simulink library "Lib_Piccolo"  (R2018b)
settings: Solver=VariableStepAuto  StartTime=0.0  StopTime=10.0  RelTol=1e-3
values from neighbouring files (symbols this model uses):
  AccelErrInt2Brakes = 0.15    [SimulationControlConfig16P.m]    (also in SimulationControlConfig16P_LEGACY.m; SimulationControlConfigTAILLESS.m = 0.2; SimulationControlConfigUTAIL.m = 0.2)
  AileronMax = 25    [SimulationControlConfig16P.m]    (also in SimulationControlConfig16P_LEGACY.m; SimulationControlConfigTAILLESS.m; SimulationControlConfigUTAIL.m)
  AileronPower = 0.00268    [SimulationControlConfig16P.m]    (also in SimulationControlConfig16P_LEGACY.m; SimulationControlConfigTAILLESS.m; SimulationControlConfigUTAIL.m)
  AileronSurfaceMax = 45    [SimulationControlConfig16P.m]    (also in SimulationControlConfig16P_LEGACY.m)
  AileronTrim = 0    [SimulationControlConfig16P.m]    (also in SimulationControlConfig16P_LEGACY.m; SimulationControlConfigTAILLESS.m; SimulationControlConfigUTAIL.m)
  Alt = 1000 + TerrainHeight    [SimulationStateConfig.m]
  AltCruise_m = testPlans(testIndx).terrainElevation * 0.3048 + 200    [SimulationControlConfig16P.m]    (also in SimulationControlConfigTAILLESS.m = 1083; SimulationControlConfigUTAIL.m = testPlans(testIndx).terrainElevation * 0.3048 + 152)
  AltitudeRate2PitchCmdIntegratorInit = 0.1    [SimulationControlPre.m]
  AltMax = 10000    [SimulationControlConfig16P.m]    (also in SimulationControlConfig16P_LEGACY.m; SimulationControlConfigTAILLESS.m; SimulationControlConfigUTAIL.m)
  AltMaxAccel = 1.25    [SimulationControlConfig16P.m]    (also in SimulationControlConfig16P_LEGACY.m = 0.9; SimulationControlConfigTAILLESS.m = 1.7; SimulationControlConfigUTAIL.m = 2)
  AltMin = 0    [SimulationControlConfig16P.m]    (also in SimulationControlConfig16P_LEGACY.m; SimulationControlConfigTAILLESS.m; SimulationControlConfigUTAIL.m)
  AltRateCmd2Pitch = 0.50    (= 0.5)    [SimulationControlConfig16P.m]    (also in SimulationControlConfig16P_LEGACY.m = 0.6; SimulationControlConfigTAILLESS.m = 0.2; SimulationControlConfigUTAIL.m = 0.3)
  AltRateError2Pitch = 0.40    (= 0.4)    [SimulationControlConfig16P.m]    (also in SimulationControlConfig16P_LEGACY.m; SimulationControlConfigTAILLESS.m = 0.55; SimulationControlConfigUTAIL.m = 0.55)
  AltRateErrorInt2Pitch = 0.50    (= 0.5)    [SimulationControlConfig16P.m]    (also in SimulationControlConfig16P_LEGACY.m = 0.45; SimulationControlConfigTAILLESS.m; SimulationControlConfigUTAIL.m = 0.75)
  AltRateLpfCutOff = 3    [SimulationControlConfig16P.m]    (also in SimulationControlConfig16P_LEGACY.m; SimulationControlConfigTAILLESS.m = 2; SimulationControlConfigUTAIL.m = 2)
  AutoNosegear2Rudder = 26    [SimulationControlConfig16P.m]    (also in SimulationControlConfig16P_LEGACY.m; SimulationControlConfigTAILLESS.m = 25.2; SimulationControlConfigUTAIL.m = 14)
  b = 5.54    [SimulationControlConfig16P.m]    (also in SimulationControlConfig16P_LEGACY.m; SimulationControlConfigTAILLESS.m = 2.37; SimulationControlConfigUTAIL.m = 2.37)
  Bank2AileronIntegratorInit = 0    [SimulationControlPre.m]
  BankMax_User = BankMax_User/180*pi    (= 0.523598775598)    [SimulationControlConfig16P.m]    (also in SimulationControlConfig16P_LEGACY.m; SimulationControlConfigTAILLESS.m = 0.610865238198; SimulationControlConfigUTAIL.m = 0.628318530718)
  baseLegFlaps = 20    [SimulationControlConfig16P.m]    (also in SimulationControlConfig16P_LEGACY.m = 0; SimulationControlConfigTAILLESS.m = 15; SimulationControlConfigUTAIL.m = 10)
  C = GeneticOpt.C    [SimulationCostFunction.m]
  c = Sw/b    (= 0.841696750903)    [SimulationControlConfig16P.m]    (also in SimulationControlConfig16P_LEGACY.m; SimulationControlConfigTAILLESS.m = 0.354008438819; SimulationControlConfigUTAIL.m = 0.354008438819)
  cell2WheelFactorMG = 5.98    [SimulationSensorConfig16P_LEGACY.m]
  cell2WheelFactorNG = 1    [SimulationSensorConfig16P_LEGACY.m]
  cellSatMaxMG = 15000    [SimulationSensorConfig16P.m]    (also in SimulationSensorConfig16P_LEGACY.m; SimulationSensorConfigTAILLESS7P.m; SimulationSensorConfigUTAIL7P.m)
  cellSatMaxNG = 1000    [SimulationSensorConfig16P.m]    (also in SimulationSensorConfig16P_LEGACY.m; SimulationSensorConfigTAILLESS7P.m; SimulationSensorConfigUTAIL7P.m)
  cellSatMinMG = -15000    [SimulationSensorConfig16P.m]    (also in SimulationSensorConfig16P_LEGACY.m; SimulationSensorConfigTAILLESS7P.m; SimulationSensorConfigUTAIL7P.m)
  cellSatMinNG = -1000    [SimulationSensorConfig16P.m]    (also in SimulationSensorConfig16P_LEGACY.m; SimulationSensorConfigTAILLESS7P.m; SimulationSensorConfigUTAIL7P.m)
  CL_Limit = CL_Max    (= 0.54)    [SimulationControlConfig16P.m]    (also in SimulationControlConfig16P_LEGACY.m; SimulationControlConfigTAILLESS.m; SimulationControlConfigUTAIL.m = 0.53)
  CL_Max = 0.54    [SimulationControlConfig16P.m]    (also in SimulationControlConfig16P_LEGACY.m; SimulationControlConfigTAILLESS.m; SimulationControlConfigUTAIL.m = 0.53)
  CL_Max_Nom = 0.465    [SimulationControlConfig16P.m]    (also in SimulationControlConfig16P_LEGACY.m; SimulationControlConfigTAILLESS.m = 0.39; SimulationControlConfigUTAIL.m)
  CL_Min = 0    [SimulationControlConfig16P.m]    (also in SimulationControlConfig16P_LEGACY.m; SimulationControlConfigTAILLESS.m; SimulationControlConfigUTAIL.m)
  ClimbMaxFraction = 0.35    [SimulationControlConfig16P.m]    (also in SimulationControlConfig16P_LEGACY.m = 0.24; SimulationControlConfigTAILLESS.m = 0.19; SimulationControlConfigUTAIL.m = 0.21)
  ClimboutMaxBank = 7.0    (= 7)    [SimulationControlConfig16P.m]    (also in SimulationControlConfig16P_LEGACY.m; SimulationControlConfigTAILLESS.m = 5; SimulationControlConfigUTAIL.m)
  ClimboutTimer = 7.0    (= 7)    [SimulationControlConfig16P.m]    (also in SimulationControlConfig16P_LEGACY.m; SimulationControlConfigTAILLESS.m; SimulationControlConfigUTAIL.m)
  dCl_per_dFlap = 0.005581818    [SimulationControlConfig16P.m]    (also in SimulationControlConfig16P_LEGACY.m = 0; SimulationControlConfigTAILLESS.m = 0; SimulationControlConfigUTAIL.m = 0)
  DecelerationCmd = 3.1    [SimulationControlConfig16P.m]    (also in SimulationControlConfig16P_LEGACY.m; SimulationControlConfigTAILLESS.m = 0.1; SimulationControlConfigUTAIL.m = 0.1)
  DeRotateLogicEndTimer = abs((NoseDownLimit_Deg-1)/DeRotateRamp_Dps)    [SimulationControlConfig16P.m]    (also in SimulationControlConfig16P_LEGACY.m; SimulationControlConfigTAILLESS.m; SimulationControlConfigUTAIL.m)
  DeRotateLogicHoldNoseUpTimer = 0.1    [SimulationControlConfig16P.m]    (also in SimulationControlConfig16P_LEGACY.m; SimulationControlConfigTAILLESS.m; SimulationControlConfigUTAIL.m)
  DeRotateLogicTimerTimeout = 2    [SimulationControlConfig16P.m]    (also in SimulationControlConfig16P_LEGACY.m; SimulationControlConfigTAILLESS.m; SimulationControlConfigUTAIL.m)
  DeRotateLowerCmdSaturation = 0    [SimulationControlConfig16P.m]    (also in SimulationControlConfig16P_LEGACY.m; SimulationControlConfigTAILLESS.m; SimulationControlConfigUTAIL.m)
  DeRotateRamp_Dps = 3    [SimulationControlConfig16P.m]    (also in SimulationControlConfig16P_LEGACY.m; SimulationControlConfigTAILLESS.m = 8; SimulationControlConfigUTAIL.m = 8)
  DeRotateUpperCmdSaturation = 7    [SimulationControlConfig16P.m]    (also in SimulationControlConfig16P_LEGACY.m; SimulationControlConfigTAILLESS.m; SimulationControlConfigUTAIL.m)
  DescentMaxFraction = 0.22    [SimulationControlConfig16P.m]    (also in SimulationControlConfig16P_LEGACY.m = 0.2; SimulationControlConfigTAILLESS.m = 0.17; SimulationControlConfigUTAIL.m = 0.17)
  DesktopSimTerrainOffset_m = 0.406    [SimulationAircraftConfig.m]
  downwindFlaps = 0    [SimulationControlConfig16P.m]    (also in SimulationControlConfig16P_LEGACY.m; SimulationControlConfigTAILLESS.m; SimulationControlConfigUTAIL.m)
  DP_init = 0.5*1.225*V_init^2    [SimulationControlConfig16P.m]    (also in SimulationControlConfig16P_LEGACY.m; SimulationControlConfigTAILLESS.m; SimulationControlConfigUTAIL.m)
  dscNoiseMG = 1    [SimulationSensorConfig16P_LEGACY.m]
  dscNoiseNG = 0.25    [SimulationSensorConfig16P_LEGACY.m]
  DSCnumBits = 24    [SimulationSensorConfig16P.m]    (also in SimulationSensorConfig16P_LEGACY.m; SimulationSensorConfigTAILLESS7P.m; SimulationSensorConfigUTAIL7P.m)
  DSCRangeMaxMG = 15000    [SimulationSensorConfig16P.m]    (also in SimulationSensorConfig16P_LEGACY.m; SimulationSensorConfigTAILLESS7P.m; SimulationSensorConfigUTAIL7P.m)
  DSCRangeMaxNG = 1000    [SimulationSensorConfig16P.m]    (also in SimulationSensorConfig16P_LEGACY.m; SimulationSensorConfigTAILLESS7P.m; SimulationSensorConfigUTAIL7P.m)
  DSCRangeMinMG = -15000    [SimulationSensorConfig16P.m]    (also in SimulationSensorConfig16P_LEGACY.m; SimulationSensorConfigTAILLESS7P.m; SimulationSensorConfigUTAIL7P.m)
  DSCRangeMinNG = -1000    [SimulationSensorConfig16P.m]    (also in SimulationSensorConfig16P_LEGACY.m; SimulationSensorConfigTAILLESS7P.m; SimulationSensorConfigUTAIL7P.m)
  dt = DLLSim.dt    [SimulationTimeStep.m]    (also in SimulationTrim.m = 0.02)
  EarlyTouchdownThreshold = 3.0    (= 3)    [SimulationControlConfig16P.m]    (also in SimulationControlConfig16P_LEGACY.m; SimulationControlConfigTAILLESS.m = 2.2; SimulationControlConfigUTAIL.m = 2.5)
  ElevatorDeflectionRate = 15    [SimulationControlConfig16P.m]    (also in SimulationControlConfig16P_LEGACY.m = 12; SimulationControlConfigTAILLESS.m = 10; SimulationControlConfigUTAIL.m = 12)
  ElevatorMax = 25    [SimulationControlConfig16P.m]    (also in SimulationControlConfig16P_LEGACY.m; SimulationControlConfigTAILLESS.m; SimulationControlConfigUTAIL.m)
  ElevatorPower = -0.002209    [SimulationControlConfig16P.m]    (also in SimulationControlConfig16P_LEGACY.m; SimulationControlConfigTAILLESS.m = -0.002956; SimulationControlConfigUTAIL.m = -0.00205983)
  ElevatorTrim = -3.5    [SimulationControlConfig16P.m]    (also in SimulationControlConfig16P_LEGACY.m; SimulationControlConfigTAILLESS.m = -6; SimulationControlConfigUTAIL.m = -8)
  elevonBias = 0    [SimulationControlConfig16P.m]    (also in SimulationControlConfig16P_LEGACY.m; SimulationControlConfigTAILLESS.m; SimulationControlConfigUTAIL.m)
  Enable_TAS_Protection = 0    [SimulationControlConfig16P.m]    (also in SimulationControlConfig16P_LEGACY.m; SimulationControlConfigTAILLESS.m; SimulationControlConfigUTAIL.m)
  EnableCrossTrackAbort = 1    [SimulationControlConfig16P.m]    (also in SimulationControlConfigTAILLESS.m; SimulationControlConfigUTAIL.m)
  EnergyBandwidth = 0.02    [SimulationControlConfig16P.m]    (also in SimulationControlConfig16P_LEGACY.m; SimulationControlConfigTAILLESS.m = 0.06; SimulationControlConfigUTAIL.m = 0.06)
  EngineLhFuelCut = 0    [SimulationAircraftConfig.m]
  EngineRhFuelCut = 0    [SimulationAircraftConfig.m]
  FastThrottleRate = 0.075    [SimulationControlConfig16P.m]    (also in SimulationControlConfig16P_LEGACY.m = 0.05; SimulationControlConfigTAILLESS.m = 0.1; SimulationControlConfigUTAIL.m = 0.1)
  FilterWarmUpTime = 2    [SimulationSensorConfig16P.m]    (also in SimulationSensorConfig16P_LEGACY.m; SimulationSensorConfigTAILLESS7P.m; SimulationSensorConfigUTAIL7P.m)
  finalApproachFlaps = 20    [SimulationControlConfig16P.m]    (also in SimulationControlConfig16P_LEGACY.m = 0; SimulationControlConfigTAILLESS.m = 22; SimulationControlConfigUTAIL.m = 10)
  FinalDescentSlope_Deg = testPlans(testIndx).descentSlope    [SimulationControlConfig16P.m]    (also in SimulationControlConfig16P_LEGACY.m; SimulationControlConfigTAILLESS.m; SimulationControlConfigUTAIL.m)
  flapMax = 0    [SimulationControlConfig16P.m]    (also in SimulationControlConfig16P_LEGACY.m; SimulationControlConfigTAILLESS.m; SimulationControlConfigUTAIL.m)
  flapRate = 7.5    [SimulationControlConfig16P.m]    (also in SimulationControlConfig16P_LEGACY.m; SimulationControlConfigTAILLESS.m = 6.6; SimulationControlConfigUTAIL.m)
  FlareHeight = 5    [SimulationControlConfig16P.m]    (also in SimulationControlConfig16P_LEGACY.m = 4.8; SimulationControlConfigTAILLESS.m = 2.5; SimulationControlConfigUTAIL.m = 2)
  FlareVerticalRate_mps = -0.4    [SimulationControlConfig16P.m]    (also in SimulationControlConfig16P_LEGACY.m = -0.5; SimulationControlConfigTAILLESS.m = -0.15; SimulationControlConfigUTAIL.m = -0.15)
  Fp_Aileron = 0.55*2*pi*RollRateLpfCutoff*dt    [SimulationControlConfig16P.m]    (also in SimulationControlConfig16P_LEGACY.m; SimulationControlConfigTAILLESS.m; SimulationControlConfigUTAIL.m)
  Fp_Alt = 0.55*AltBandwidth    (= 0.099)    [SimulationControlConfig16P.m]    (also in SimulationControlConfig16P_LEGACY.m; SimulationControlConfigTAILLESS.m = 0.587477826221; SimulationControlConfigUTAIL.m = 0.69115038379)
  Fp_AltRate = 0.55*2*pi*AltRateLpfCutOff*dt    [SimulationControlConfig16P.m]    (also in SimulationControlConfig16P_LEGACY.m; SimulationControlConfigTAILLESS.m; SimulationControlConfigUTAIL.m)
  Fp_Elevator = 0.55*2*pi*PitchRateLpfCutoff*dt    [SimulationControlConfig16P.m]    (also in SimulationControlConfig16P_LEGACY.m; SimulationControlConfigTAILLESS.m; SimulationControlConfigUTAIL.m)
  Fp_Energy = 0.55*2*pi*EnergyBandwidth    (= 0.069115038379)    [SimulationControlConfig16P.m]    (also in SimulationControlConfig16P_LEGACY.m; SimulationControlConfigTAILLESS.m = 0.207345115137; SimulationControlConfigUTAIL.m = 0.207345115137)
  Fp_Energy2 = 0.55*2*pi*EnergyBandwidth*dt    [SimulationControlConfig16P.m]    (also in SimulationControlConfig16P_LEGACY.m; SimulationControlConfigTAILLESS.m; SimulationControlConfigUTAIL.m)
  Fp_Pitch = 0.55*2*pi*PitchBandwidth    (= 2.76460153516)    [SimulationControlConfig16P.m]    (also in SimulationControlConfig16P_LEGACY.m = 3.11017672705; SimulationControlConfigTAILLESS.m = 3.80132711084; SimulationControlConfigUTAIL.m = 2.41902634326)
  Fp_Pitch_2 = 0.55*2*pi*PitchBandwidth*dt    [SimulationControlConfig16P.m]    (also in SimulationControlConfig16P_LEGACY.m; SimulationControlConfigTAILLESS.m; SimulationControlConfigUTAIL.m)
  Fp_Roll = RollBandwidth^2    (= 1)    [SimulationControlConfig16P.m]    (also in SimulationControlConfig16P_LEGACY.m = 1.44; SimulationControlConfigTAILLESS.m; SimulationControlConfigUTAIL.m)
  Fp_Rudder = 0.55*2*pi*YawRateLpfCutoff*dt    [SimulationControlConfig16P.m]    (also in SimulationControlConfig16P_LEGACY.m; SimulationControlConfigTAILLESS.m; SimulationControlConfigUTAIL.m)
  Fp_TAS = 0.55*2*pi*TASBandwidth    (= 0.103672557568)    [SimulationControlConfig16P.m]    (also in SimulationControlConfig16P_LEGACY.m; SimulationControlConfigTAILLESS.m = 0.172787595947; SimulationControlConfigUTAIL.m = 0.172787595947)
  Fp_TAS_Filter = 2*pi*TasLpfCutoff*dt    [SimulationControlConfig16P.m]    (also in SimulationControlConfig16P_LEGACY.m; SimulationControlConfigTAILLESS.m; SimulationControlConfigUTAIL.m)
  Fp_Turn = 0.55*2*pi*TurnErrLPFcutoff    (= 0.0345575191895)    [SimulationControlConfig16P.m]    (also in SimulationControlConfig16P_LEGACY.m; SimulationControlConfigTAILLESS.m = 0.172787595947; SimulationControlConfigUTAIL.m = 0.172787595947)
  Fp_TurnDerr = 0.55*2*pi*TurnDerivativeLPFcutoff    (= 0.0345575191895)    [SimulationControlConfig16P.m]    (also in SimulationControlConfig16P_LEGACY.m; SimulationControlConfigTAILLESS.m = 0.172787595947; SimulationControlConfigUTAIL.m = 0.172787595947)
  FTV = 3    [SimulationAircraftConfig.m]
  ftvStaticPositionError = 1/1.18    (= 0.847457627119)    [SimulationSensorConfig16P.m]    (also in SimulationSensorConfig16P_LEGACY.m; SimulationSensorConfigTAILLESS7P.m = 1; SimulationSensorConfigUTAIL7P.m = 1)
  g = 9.81    [SimulationStateConfig.m]
  GustSpd_Kts = testPlans(testIndx).gustSpd    [SimulationStateConfig.m]
  GustTriggerVal = testPlans(testIndx).gustTriggerVal    [SimulationStateConfig.m]
  HeadingErr2TurnRate = 0.5    [SimulationControlConfig16P.m]    (also in SimulationControlConfig16P_LEGACY.m; SimulationControlConfigTAILLESS.m; SimulationControlConfigUTAIL.m)
  HeadingErrDer2TurnRate = 0.3    [SimulationControlConfig16P.m]    (also in SimulationControlConfig16P_LEGACY.m; SimulationControlConfigTAILLESS.m; SimulationControlConfigUTAIL.m)
  IASbounce = IASstall*0.8    [SimulationControlPre.m]
  IAScruiseCMD = sqrt(2*m*9.81/(1.225*Sw*CL_cruise))    [SimulationControlConfig16P.m]    (also in SimulationControlConfig16P_LEGACY.m; SimulationControlConfigTAILLESS.m; SimulationControlConfigUTAIL.m)
  IASfinalCMD = 1.12 * IASmin    [SimulationControlConfig16P.m]    (also in SimulationControlConfig16P_LEGACY.m = 1.10 * IASmin; SimulationControlConfigTAILLESS.m = 1.10 * IASmin; SimulationControlConfigUTAIL.m = 1.15 * IASmin)
  IASflareCMD = IASstall    [SimulationControlConfig16P.m]    (also in SimulationControlConfig16P_LEGACY.m; SimulationControlConfigTAILLESS.m; SimulationControlConfigUTAIL.m)
  IASmax = 64    [SimulationControlConfig16P.m]    (also in SimulationControlConfig16P_LEGACY.m = 46; SimulationControlConfigTAILLESS.m = 38.58; SimulationControlConfigUTAIL.m = 35)
  IASmin = sqrt(2*m*9.81/(1.225*Sw*0.9*CL_Max_Nom))    [SimulationControlConfig16P.m]    (also in SimulationControlConfig16P_LEGACY.m; SimulationControlConfigTAILLESS.m; SimulationControlConfigUTAIL.m)
  IASshortCMD = IASstall    [SimulationControlConfig16P.m]    (also in SimulationControlConfig16P_LEGACY.m; SimulationControlConfigTAILLESS.m; SimulationControlConfigUTAIL.m)
  IASstall = sqrt(2*m*9.81/(1.225*Sw*CL_Max))    [SimulationControlConfig16P.m]    (also in SimulationControlConfig16P_LEGACY.m; SimulationControlConfigTAILLESS.m; SimulationControlConfigUTAIL.m)
  inFlight = 1    [SimulationControlConfig16P.m]    (also in SimulationControlConfigTAILLESS.m; SimulationControlConfigUTAIL.m)
  JetCatOffset = 5    [SimulationControlConfig16P.m]    (also in SimulationControlConfig16P_LEGACY.m)
  LaunchRollingElevator = -1.5    [SimulationControlConfig16P.m]    (also in SimulationControlConfig16P_LEGACY.m; SimulationControlConfigTAILLESS.m = 1; SimulationControlConfigUTAIL.m = 1)
  ldg_NosegearMax = 10    [SimulationControlConfig16P.m]    (also in SimulationControlConfig16P_LEGACY.m; SimulationControlConfigTAILLESS.m; SimulationControlConfigUTAIL.m)
  ldg_TrackVyErrInt2Nosegear = 0.1250    (= 0.125)    [SimulationControlConfig16P.m]    (also in SimulationControlConfig16P_LEGACY.m; SimulationControlConfigTAILLESS.m = 0.00714285714286; SimulationControlConfigUTAIL.m = 0.00714285714286)
  ldg_TrackVyErrPro2Nosegear = 0.35    [SimulationControlConfig16P.m]    (also in SimulationControlConfig16P_LEGACY.m; SimulationControlConfigTAILLESS.m = 0.0546666666667; SimulationControlConfigUTAIL.m = 0.0546666666667)
  ldg_TrackY2Vy = 0.07    [SimulationControlConfig16P.m]    (also in SimulationControlConfig16P_LEGACY.m; SimulationControlConfigTAILLESS.m = 0.17; SimulationControlConfigUTAIL.m = 0.17)
  ldg_Vy2NosegearScalingPower = 1.075    [SimulationControlConfig16P.m]    (also in SimulationControlConfig16P_LEGACY.m; SimulationControlConfigTAILLESS.m = 0.6; SimulationControlConfigUTAIL.m = 0.5)
  ldg_Y2VyScalingPower = 0.175    [SimulationControlConfig16P.m]    (also in SimulationControlConfig16P_LEGACY.m; SimulationControlConfigTAILLESS.m = 0; SimulationControlConfigUTAIL.m = 0)
  ldg_YawRate2Nosegear = 0.175    [SimulationControlConfig16P.m]    (also in SimulationControlConfig16P_LEGACY.m; SimulationControlConfigTAILLESS.m = 0.065; SimulationControlConfigUTAIL.m = 0.065)
  LiftSlope = 0.064285    [SimulationControlConfig16P.m]    (also in SimulationControlConfig16P_LEGACY.m; SimulationControlConfigTAILLESS.m = 0.058631; SimulationControlConfigUTAIL.m)
  LPFaileronInit = 0    [SimulationControlPre.m]
  LPFclestInit = 0    [SimulationControlPre.m]
  LPFenergyFFInit = 0    [SimulationControlPre.m]
  LPFtasInit = V_init + 2    [SimulationControlPre.m]
  LPFthrottleInit = ThrottleTrim    [SimulationControlPre.m]
  LPFturnErrInit = 0    [SimulationControlPre.m]
  ... (+115 more)
undefined symbols (not defined in the file or in its folder): abortFlag, alphaHPF, apmDelay, BRWNOUT, CRAWOR, CRAWUR, DiscIntNeverNeededParam, DLLSim, DLLSimStep, ECOMOR, ECOMUR, Fp_Tas, GustTrigger_HeightAgl_m, IPSTAT, LCINTEG, Ldg_Persist_Time, LOWER_FLAGS, MSG_ENABLE, NoiseStd, OLDVAL, OVERRIDE_ENABLE, OVERRIDE_VALUE, REBOOT, reversionEnable, revIASMax, revIASMin, revPitchMax, revPitchMin, revPitchRateMax, revRollMax, revRollRateMax, SAMPLE, SCALON, SensorModel, sigbuilder_block, Sim_Vx, Sim_Vy, Sim_Vz, Sim_Xpos, Sim_Ypos, Sim_Zpos, SYSOR, SYSUR, TARE, TEMPOR, TEMPUR, testIndx, testPlan, testPlans, Trim_piccoloInCmd, Trim_REFSI_FD_IN_nmodeCgShifterCmd_Ft, Trim_REFSI_FD_IN_nmodeFlapLhIBCmd_Deg, Trim_REFSI_FD_IN_nmodeFlapLhOBCmd_Deg, Trim_REFSI_FD_IN_nmodeFlapRhIBCmd_Deg, Trim_REFSI_FD_IN_nmodeFlapRhOBCmd_Deg, Trim_REFSI_FD_IN_nmodeSlatLhCmd_Deg, Trim_REFSI_FD_IN_nmodeSlatRhCmd_Deg, Trim_REFSI_FD_IN_nmodeSplrLhInbdCmd_Deg, Trim_REFSI_FD_IN_nmodeSplrLhOutbdCmd_Deg ... (+5)
libraries: simulink x866, aerolibconvert2 x60, $bdroot x52, aerolibatmos2 x5, dspswit3 x5, simulink_extras x4, dsparch4 x2, Lib_Piccolo_Alt x2, eeGeneralControl x1, dspindex x1
(part 34 of 44)

== system Lib_Piccolo/Ground Detection Systems/WoW Wrapper/Variant Subsystem/Load Cell WoW Model 1 7P AsFlown/LPF N ==
  Input : Inport
  Reset : Inport  Port=2
  Add1 : Sum  Inputs=++|
  Compare To Constant2 : simulink/Logic and Bit Operations/Compare To Constant  relop=>  const=0  OutDataTypeStr=uint8
  Constant11 : Constant  Value=2
  Switch1 : Switch  Criteria=u2 > Threshold
  Unit Delay1 : UnitDelay  InitialCondition=Init  SampleTime=-1
  a1 : Gain  Gain=1-0.221168
  b0 : Gain  Gain=0.221168
  Output : Outport
  wires:
  Constant11/1 -> Compare To Constant2/1
  Compare To Constant2/1 -> Switch1/2
  Switch1/1 -> Output/1
  Input/1 -> b0/1, Switch1/3
  a1/1 -> Add1/1
  Add1/1 -> Switch1/1, Unit Delay1/1
  b0/1 -> Add1/2
  Unit Delay1/1 -> a1/1

== system Lib_Piccolo/Ground Detection Systems/WoW Wrapper/Variant Subsystem/Load Cell WoW Model 1 7P AsFlown/LPF R ==
  Input : Inport
  Reset : Inport  Port=2
  Add1 : Sum  Inputs=++|
  Compare To Constant2 : simulink/Logic and Bit Operations/Compare To Constant  relop=>  const=0  OutDataTypeStr=uint8
  Constant11 : Constant  Value=2
  Switch1 : Switch  Criteria=u2 > Threshold
  Unit Delay1 : UnitDelay  InitialCondition=Init  SampleTime=-1
  a1 : Gain  Gain=1-0.221168
  b0 : Gain  Gain=0.221168
  Output : Outport
  wires:
  Constant11/1 -> Compare To Constant2/1
  Compare To Constant2/1 -> Switch1/2
  Switch1/1 -> Output/1
  Input/1 -> b0/1, Switch1/3
  a1/1 -> Add1/1
  Add1/1 -> Switch1/1, Unit Delay1/1
  b0/1 -> Add1/2
  Unit Delay1/1 -> a1/1

== system Lib_Piccolo/Ground Detection Systems/WoW Wrapper/Variant Subsystem/Load Cell WoW Model 1 7P AsFlown/Landing Configuration ==
  Sim.WOW_Filt : Inport
  AND : Logic  IconShape=distinctive  AllPortsSameDT=off  OutDataTypeStr=boolean
  Bus Selector : BusSelector  OutputSignals=Sim:WOW_Filt_NG,Sim:WOW_Filt_L,Sim:WOW_Filt_R
  Gain1 : Gain
  Gain2 : Gain
  Hysteresis L : Relay  OnSwitchValue=Ldg_Load_Thresh_Upper  OffSwitchValue=Ldg_Load_Thresh_Lower
  Hysteresis R : Relay  OnSwitchValue=Ldg_Load_Thresh_Upper  OffSwitchValue=Ldg_Load_Thresh_Lower
  Latch : Subsystem
  Latch Timer Selection : Subsystem
  Persistance Timer : Subsystem  mask{period=Ldg_Persist_Time}
      mask prompts: period "Period [s]"
  Terminator : Terminator
  Terminator1 : Terminator
  Terminator2 : Terminator
  ContactBool : Outport
  wires:
  Persistance Timer/1(Expired) -> Latch/1(D)
  Hysteresis L/1 -> AND/1, Gain1/1
  Hysteresis R/1 -> AND/2, Gain2/1
  Gain1/1 -> Terminator1/1  "ContactL"
  Gain2/1 -> Terminator2/1  "ContactR"
  Latch/1(Q_Latched) -> Latch Timer Selection/1(ContactBool), ContactBool/1  "ContactBool"
  Sim.WOW_Filt/1 -> Bus Selector/1
  Bus Selector/1 -> Terminator/1  "<Sim:WOW_Filt_NG>"
  Bus Selector/2 -> Hysteresis L/1  "<Sim:WOW_Filt_L>"
  Bus Selector/3 -> Hysteresis R/1  "<Sim:WOW_Filt_R>"
  AND/1 -> Persistance Timer/1(Enable/!Rst)
  Latch Timer Selection/1(switchedTimer) -> Latch/2(Enable/!Rst)

== system Lib_Piccolo/Ground Detection Systems/WoW Wrapper/Variant Subsystem/Load Cell WoW Model 1 7P AsFlown/T//O Configuration ==
  note: Unlike when landing our persistance and latching is inverted relative to Weight Off both gears.
      |
      | Protection against WOW Failure. In the Event of a Sensor Failure and AC lift's off, NZ threshold overides WOW signal.
  Sim.WOW_Filt : Inport
  AND : Logic  IconShape=distinctive  AllPortsSameDT=off  OutDataTypeStr=boolean
  Bus Selector : BusSelector  OutputSignals=Sim:WOW_Filt_NG,Sim:WOW_Filt_L,Sim:WOW_Filt_R
  Compare To Constant1 : simulink/Logic and Bit Operations/Compare To Constant  relop=<  const=TO_Load_Thresh  OutDataTypeStr=uint8
  Compare To Constant2 : simulink/Logic and Bit Operations/Compare To Constant  relop=<  const=TO_Load_Thresh  OutDataTypeStr=uint8
  Latch : Subsystem
  Latch Timer : Subsystem  mask{period=TO_Latch_Time}
      mask prompts: period "Period [s]"
  NOT : Logic  Operator=NOT  IconShape=distinctive  AllPortsSameDT=off  OutDataTypeStr=boolean
  NOT2 : Logic  Operator=NOT  IconShape=distinctive  AllPortsSameDT=off  OutDataTypeStr=boolean
  Persistance Timer : Subsystem  mask{period=TO_Persist_Time}
      mask prompts: period "Period [s]"
  Terminator : Terminator
  Unit Delay : UnitDelay  SampleTime=-1
  ContactBool : Outport
  wires:
  Bus Selector/3 -> Compare To Constant1/1  "<Sim:WOW_Filt_R>"
  Bus Selector/2 -> Compare To Constant2/1  "<Sim:WOW_Filt_L>"
  Bus Selector/1 -> Terminator/1  "<Sim:WOW_Filt_NG>"
  Sim.WOW_Filt/1 -> Bus Selector/1
  NOT/1 -> Latch/2(Enable/!Rst)
  Latch/1(Q_Latched) -> NOT2/1, Unit Delay/1  "ContactBool"
  AND/1 -> Persistance Timer/1(Enable/!Rst)
  Compare To Constant1/1 -> AND/2
  Unit Delay/1 -> Latch Timer/1(Enable/!Rst)
  Latch Timer/1(Expired) -> NOT/1
  Compare To Constant2/1 -> AND/1
  Persistance Timer/1(Expired) -> Latch/1(D)
  NOT2/1 -> ContactBool/1

== system Lib_Piccolo/Ground Detection Systems/WoW Wrapper/Variant Subsystem/Load Cell WoW Model 16/Subsystem ==
  note: Ground Detection Logic
  Sim.WOW_NG_N : Inport
  Sim.WOW_L_N : Inport  Port=2
  RESET : Inport  Port=3
  Sim.WOW_R_N : Inport  Port=4
  PICCOLO_AP_MODE : Inport  Port=5
  Bus Creator1 : BusCreator  Inputs=3
  Compare To Constant1 : simulink/Logic and Bit Operations/Compare To Constant  relop===  const=0  OutDataTypeStr=uint8
  Compare To Constant6 : simulink/Logic and Bit Operations/Compare To Constant  relop=>=  const=4  OutDataTypeStr=uint8
  LPF L : Subsystem  mask{Cutoff=SensorModel.WOW.Cell.fc, Init=0}
      mask prompts: Cutoff "Cutoff Frequency [Hz]"; Init "Initial Condition"
  LPF N : Subsystem  mask{Cutoff=SensorModel.WOW.Cell.fc, Init=0}
      mask prompts: Cutoff "Cutoff Frequency [Hz]"; Init "Initial Condition"
  LPF R : Subsystem  mask{Cutoff=SensorModel.WOW.Cell.fc, Init=0}
      mask prompts: Cutoff "Cutoff Frequency [Hz]"; Init "Initial Condition"
  Landing Configuration : Subsystem
  OR : Logic  Operator=OR  IconShape=distinctive  AllPortsSameDT=off  OutDataTypeStr=boolean
  Saturation : Saturate  UpperLimit=SensorModel.WOW.Cell.SaturationUpper  LowerLimit=SensorModel.WOW.Cell.SaturationLower
  Saturation1 : Saturate  UpperLimit=SensorModel.WOW.Cell.SaturationUpper  LowerLimit=SensorModel.WOW.Cell.SaturationLower
  Saturation2 : Saturate  UpperLimit=SensorModel.WOW.Cell.SaturationUpper  LowerLimit=SensorModel.WOW.Cell.SaturationLower
  Switch : Switch  Criteria=u2 > Threshold
  T/O Configuration : Subsystem
  Sim.WOW_Filt_NG : Outport
  Sim.WOW_Filt_L : Outport  Port=2
  Contact : Outport  Port=3
  Sim.WOW_Filt_R : Outport  Port=4
  wires:
  Sim.WOW_R_N/1 -> Saturation2/1
  Switch/1 -> Contact/1
  OR/1 -> Switch/2
  T/O Configuration/1(ContactBool) -> Switch/3
  Compare To Constant1/1 -> OR/2
  LPF N/1(Output) -> Bus Creator1/1, Sim.WOW_Filt_NG/1  "Sim.WOW_Filt_NG"
  Landing Configuration/1(ContactBool) -> Switch/1
  Sim.WOW_NG_N/1 -> Saturation/1
  RESET/1 -> LPF R/2(Reset), LPF L/2(Reset), LPF N/2(Reset)
  Sim.WOW_L_N/1 -> Saturation1/1
  LPF L/1(Output) -> Bus Creator1/2, Sim.WOW_Filt_L/1  "Sim.WOW_Filt_L"
  Bus Creator1/1 -> Landing Configuration/1(Sim.WOW_Filt), T/O Configuration/1(Sim.WOW_Filt)
  Compare To Constant6/1 -> OR/1
  PICCOLO_AP_MODE/1 -> Compare To Constant6/1, Compare To Constant1/1
  LPF R/1(Output) -> Bus Creator1/3, Sim.WOW_Filt_R/1  "Sim.WOW_Filt_R"
  Saturation2/1 -> LPF R/1(Input)
  Saturation1/1 -> LPF L/1(Input)
  Saturation/1 -> LPF N/1(Input)

== system Lib_Piccolo/Ground Detection Systems/WoW Wrapper/Variant Subsystem/Load Cell WoW Model 18/Conversion - NG ==
  Lbf : Inport
  Lbf2N : Gain  Gain=4.44822
  N : Outport
  wires:
  Lbf/1 -> Lbf2N/1
  Lbf2N/1 -> N/1

== system Lib_Piccolo/Ground Detection Systems/WoW Wrapper/Variant Subsystem/Load Cell WoW Model 18/Subsystem ==
  note: Ground Detection Logic
  WOW_NG_N : Inport
  WOW_MGL_N : Inport  Port=2
  WOW_MGR_N : Inport  Port=3
  RESET : Inport  Port=4
  PICCOLO_AP_MODE : Inport  Port=5
  MGR_DSC_FAIL : Inport  Port=6  OutDataTypeStr=uint8
  MGL_DSC_FAIL : Inport  Port=7  OutDataTypeStr=uint8
  AND1 : Logic  IconShape=distinctive  AllPortsSameDT=off
  Bus Creator1 : BusCreator  Inputs=3
  Bus Creator2 : BusCreator  Inputs=2
  Compare To Constant1 : simulink/Logic and Bit Operations/Compare To Constant  relop===  const=0  OutDataTypeStr=uint8
  Compare To Constant6 : simulink/Logic and Bit Operations/Compare To Constant  relop=>=  const=4  OutDataTypeStr=uint8
  Data Type Conversion : DataTypeConversion  OutDataTypeStr=uint8
  LPF L : Subsystem  mask{Cutoff=SensorModel.WOW.Cell.fc, Init=0}
      mask prompts: Cutoff "Cutoff Frequency [Hz]"; Init "Initial Condition"
  LPF N : Subsystem  mask{Cutoff=SensorModel.WOW.Cell.fc, Init=0}
      mask prompts: Cutoff "Cutoff Frequency [Hz]"; Init "Initial Condition"
  LPF R : Subsystem  mask{Cutoff=SensorModel.WOW.Cell.fc, Init=0}
      mask prompts: Cutoff "Cutoff Frequency [Hz]"; Init "Initial Condition"
  Landing Configuration : Subsystem
  OR : Logic  Operator=OR  IconShape=distinctive  AllPortsSameDT=off  OutDataTypeStr=boolean
  Saturation : Saturate  UpperLimit=SensorModel.WOW.Cell.SaturationUpper  LowerLimit=SensorModel.WOW.Cell.SaturationLower
  Saturation1 : Saturate  UpperLimit=SensorModel.WOW.Cell.SaturationUpper  LowerLimit=SensorModel.WOW.Cell.SaturationLower
  Saturation2 : Saturate  UpperLimit=SensorModel.WOW.Cell.SaturationUpper  LowerLimit=SensorModel.WOW.Cell.SaturationLower
  Switch : Switch  Criteria=u2 > Threshold
  T/O Configuration : Subsystem
  WOW_Filt_NG_N : Outport
  WOW_Filt_MGL_N : Outport  Port=2
  WOW_Filt_MGR_N : Outport  Port=3
  Contact : Outport  Port=4  OutDataTypeStr=uint8
  WOW_Logic_Disable : Outport  Port=5  OutDataTypeStr=uint8
  wires:
  WOW_MGR_N/1 -> Saturation2/1
  Switch/1 -> Contact/1
  OR/1 -> Switch/2
  T/O Configuration/1(ContactBool) -> Switch/3
  Compare To Constant1/1 -> OR/2
  LPF N/1(Output) -> Bus Creator1/1, WOW_Filt_NG_N/1  "WOW_Filt_NG_N"
  Landing Configuration/1(ContactBool) -> Switch/1
  WOW_NG_N/1 -> Saturation/1
  RESET/1 -> LPF R/2(Reset), LPF L/2(Reset), LPF N/2(Reset)
  WOW_MGL_N/1 -> Saturation1/1
  LPF L/1(Output) -> Bus Creator1/2, WOW_Filt_MGL_N/1  "WOW_Filt_MGL_N"
  Bus Creator1/1 -> Landing Configuration/1(WOW_Filt), T/O Configuration/1(WOW_Filt)
  Compare To Constant6/1 -> OR/1
  PICCOLO_AP_MODE/1 -> Compare To Constant6/1, Compare To Constant1/1
  LPF R/1(Output) -> Bus Creator1/3, WOW_Filt_MGR_N/1  "WOW_Filt_MGR_N"
  Saturation2/1 -> LPF R/1(Input)
  Saturation1/1 -> LPF L/1(Input)
  Saturation/1 -> LPF N/1(Input)
  MGL_DSC_FAIL/1 -> AND1/1, Bus Creator2/2  "MGL_DSC_FAIL"
  MGR_DSC_FAIL/1 -> AND1/2, Bus Creator2/1  "MGR_DSC_FAIL"
  Bus Creator2/1 -> Landing Configuration/2(DSC_Fail), T/O Configuration/2(DSC_Fail)
  AND1/1 -> Data Type Conversion/1  "LogicDisable"
  Data Type Conversion/1 -> WOW_Logic_Disable/1

== system Lib_Piccolo/Ground Detection Systems/WoW Wrapper/Variant Subsystem/Load Cell WoW Model 20/Bus Formatting MGL ==
  WOW_N : Inport
  Bus Creator2 : BusCreator  Inputs=6  OutDataTypeStr=Bus: GEAR_INPUT_BUS  NonVirtualBus=on
  FLAG : Constant  Value=SensorModel.WOW.Cell.MGL_FAIL  OutDataTypeStr=uint16
  STALE_FLAGS : Constant  Value=0  OutDataTypeStr=boolean
  STALE_LOAD : Constant  Value=0  OutDataTypeStr=boolean
  STAT : Constant  Value=0  OutDataTypeStr=uint16
  TARE VALUE : Constant  Value=0  OutDataTypeStr=single
  Bus Out : Outport
  wires:
  TARE VALUE/1 -> Bus Creator2/2  "TARE_N"
  STALE_FLAGS/1 -> Bus Creator2/6  "STALE_FLAGS"
  WOW_N/1 -> Bus Creator2/1  "WOW_N"
  Bus Creator2/1 -> Bus Out/1
  STAT/1 -> Bus Creator2/4  "DSC_STAT_WORD"
  FLAG/1 -> Bus Creator2/3  "DSC_FLAG_WORD"
  STALE_LOAD/1 -> Bus Creator2/5  "STALE_LOAD"

== system Lib_Piccolo/Ground Detection Systems/WoW Wrapper/Variant Subsystem/Load Cell WoW Model 20/Bus Formatting MGR ==
  WOW_N : Inport
  Bus Creator2 : BusCreator  Inputs=6  OutDataTypeStr=Bus: GEAR_INPUT_BUS  NonVirtualBus=on
  FLAG : Constant  Value=SensorModel.WOW.Cell.MGR_FAIL  OutDataTypeStr=uint16
  STALE_FLAGS : Constant  Value=0  OutDataTypeStr=boolean
  STALE_LOAD : Constant  Value=0  OutDataTypeStr=boolean
  STAT : Constant  Value=0  OutDataTypeStr=uint16
  TARE VALUE : Constant  Value=0  OutDataTypeStr=single
  Bus Out : Outport
  wires:
  TARE VALUE/1 -> Bus Creator2/2  "TARE_N"
  STALE_FLAGS/1 -> Bus Creator2/6  "STALE_FLAGS"
  WOW_N/1 -> Bus Creator2/1  "WOW_N"
  Bus Creator2/1 -> Bus Out/1
  STAT/1 -> Bus Creator2/4  "DSC_STAT_WORD"
  FLAG/1 -> Bus Creator2/3  "DSC_FLAG_WORD"
  STALE_LOAD/1 -> Bus Creator2/5  "STALE_LOAD"

== system Lib_Piccolo/Ground Detection Systems/WoW Wrapper/Variant Subsystem/Load Cell WoW Model 20/Bus Formatting NG ==
  WOW_N : Inport
  Bus Creator2 : BusCreator  Inputs=6  OutDataTypeStr=Bus: GEAR_INPUT_BUS  NonVirtualBus=on
  FLAG : Constant  Value=0  OutDataTypeStr=uint16
  STALE_FLAGS : Constant  Value=0  OutDataTypeStr=boolean
  STALE_LOAD : Constant  Value=0  OutDataTypeStr=boolean
  STAT : Constant  Value=0  OutDataTypeStr=uint16
  TARE VALUE : Constant  Value=0  OutDataTypeStr=single
  Bus Out : Outport
  wires:
  STALE_LOAD/1 -> Bus Creator2/5  "STALE_LOAD"
  FLAG/1 -> Bus Creator2/3  "DSC_FLAG_WORD"
  STAT/1 -> Bus Creator2/4  "DSC_STAT_WORD"
  Bus Creator2/1 -> Bus Out/1
  WOW_N/1 -> Bus Creator2/1  "WOW_N"
  STALE_FLAGS/1 -> Bus Creator2/6  "STALE_FLAGS"
  TARE VALUE/1 -> Bus Creator2/2  "TARE_N"

== system Lib_Piccolo/Ground Detection Systems/WoW Wrapper/Variant Subsystem/Load Cell WoW Model 20/DSC Data Acquisition ==
  NG Cell Load N : Inport
  MGL Cell Load N : Inport  Port=2
  MGR Cell Load N : Inport  Port=3
  DSC Noise L : RandomNumber  Variance=(SensorModel.WOW.Cell.dscNoiseMG/6)^2  Seed=20  SampleTime=dt
  DSC Noise N : RandomNumber  Variance=(SensorModel.WOW.Cell.dscNoiseNG/6)^2  Seed=10  SampleTime=dt
  DSC Noise R : RandomNumber  Variance=(SensorModel.WOW.Cell.dscNoiseMG/6)^2  Seed=30  SampleTime=dt
  Data Type L : DataTypeConversion  OutDataTypeStr=single
  Data Type N : DataTypeConversion  OutDataTypeStr=single
  Data Type R : DataTypeConversion  OutDataTypeStr=single
  Quantization L : Quantizer  QuantizationInterval=(SensorModel.WOW.Cell.calibrationSlopeMG * (SensorModel.WOW.Cell.fullScaleRange/SensorModel.WOW.Cell.effectiveCounts))
  Quantization N : Quantizer  QuantizationInterval=(SensorModel.WOW.Cell.calibrationSlopeNG * (SensorModel.WOW.Cell.fullScaleRange/SensorModel.WOW.Cell.effectiveCounts))
  Quantization R : Quantizer  QuantizationInterval=(SensorModel.WOW.Cell.calibrationSlopeMG * (SensorModel.WOW.Cell.fullScaleRange/SensorModel.WOW.Cell.effectiveCounts))
  Sum : Sum  Inputs=|++
  Sum1 : Sum  Inputs=|++
  Sum2 : Sum  Inputs=|++
  NG DSC Load N : Outport  VectorParamsAs1DForOutWhenUnconnected=on
  MGL DSC Load N : Outport  Port=2  VectorParamsAs1DForOutWhenUnconnected=on
  MGR DSC Load N : Outport  Port=3  VectorParamsAs1DForOutWhenUnconnected=on
  wires:
  NG Cell Load N/1 -> Sum2/1
  DSC Noise L/1 -> Sum/2
  Sum1/1 -> Quantization R/1
  DSC Noise N/1 -> Sum2/2
  DSC Noise R/1 -> Sum1/2
  Sum2/1 -> Quantization N/1
  Sum/1 -> Quantization L/1
  MGR Cell Load N/1 -> Sum1/1
  Quantization N/1 -> Data Type N/1
  Quantization L/1 -> Data Type L/1
  Quantization R/1 -> Data Type R/1
  Data Type N/1 -> NG DSC Load N/1
  Data Type L/1 -> MGL DSC Load N/1
  Data Type R/1 -> MGR DSC Load N/1
  MGL Cell Load N/1 -> Sum/1

== system Lib_Piccolo/Ground Detection Systems/WoW Wrapper/Variant Subsystem/Load Cell WoW Model 20/Load Cell and Unit Conversion ==
  NG Wheel Load Lbf : Inport
  MGL Wheel Load Lbf : Inport  Port=2
  MGR Wheel Load Lbf : Inport  Port=3
  Conversion - MGL : Subsystem
  Conversion - MGR : Subsystem
  Conversion - NG : Subsystem
  Wheel-to-Cell Scaling MGL : Subsystem  mask{polyA=SensorModel.WOW.Cell.polyA.inverseMGL, polyB=SensorModel.WOW.Cell.polyB.inverseMGL, polyC=SensorModel.WOW.Cell.polyC.inverseMGL}
      mask prompts: polyA "Inverse Polynomial Coefficient A"; polyB "Inverse Polynomial Coefficient B"; polyC "Inverse Polynomial Coefficient C"
      mask DialogControl DescTextVar Prompt: Invserse polynomial to produce approximate loads as seen by the load cell, due to linkages and other mechanical factors.
  Wheel-to-Cell Scaling MGR : Subsystem  mask{polyA=SensorModel.WOW.Cell.polyA.inverseMGR, polyB=SensorModel.WOW.Cell.polyB.inverseMGR, polyC=SensorModel.WOW.Cell.polyC.inverseMGR}
      mask prompts: polyA "Inverse Polynomial A"; polyB "Inverse Polynomial B"; polyC "Inverse Polynomial C"
      mask DialogControl DescTextVar Prompt: Invserse polynomial to produce approximate loads as seen by the load cell, due to linkages and other mechanical factors.
  Wheel-to-Cell Scaling NG : Subsystem  mask{polyA=SensorModel.WOW.Cell.polyA.inverseNG, polyB=SensorModel.WOW.Cell.polyB.inverseNG, polyC=SensorModel.WOW.Cell.polyC.inverseNG}
      mask prompts: polyA "Inverse Polynomial Coefficient A"; polyB "Inverse Polynomial Coefficient B"; polyC "Inverse Polynomial Coefficient C"
      mask DialogControl DescTextVar Prompt: Invserse polynomial to produce approximate loads as seen by the load cell, due to linkages and other mechanical factors.
  NG Cell Load N : Outport  VectorParamsAs1DForOutWhenUnconnected=on
  MGL Cell Load N : Outport  Port=2  VectorParamsAs1DForOutWhenUnconnected=on
  MGR Cell Load N : Outport  Port=3  VectorParamsAs1DForOutWhenUnconnected=on
  wires:
  Wheel-to-Cell Scaling MGR/1(Cell Load N) -> MGR Cell Load N/1
  Conversion - NG/1(N) -> Wheel-to-Cell Scaling NG/1(Wheel Load N)
  MGR Wheel Load Lbf/1 -> Conversion - MGR/1(Lbf)
  Conversion - MGL/1(N) -> Wheel-to-Cell Scaling MGL/1(Wheel Load N)
  Wheel-to-Cell Scaling MGL/1(Cell Load N) -> MGL Cell Load N/1
  Conversion - MGR/1(N) -> Wheel-to-Cell Scaling MGR/1(Wheel Load N)
  Wheel-to-Cell Scaling NG/1(Cell Load N) -> NG Cell Load N/1
  MGL Wheel Load Lbf/1 -> Conversion - MGL/1(Lbf)
  NG Wheel Load Lbf/1 -> Conversion - NG/1(Lbf)

== system Lib_Piccolo/Ground Detection Systems/WoW Wrapper/Variant Subsystem/Load Cell WoW Model 20/Subsystem ==
  Bus Creator : BusCreator  Inputs=SAMPLE,TARE,MSG_ENABLE,OVERRIDE_ENABLE,OVERRIDE_VALUE  OutDataTypeStr=Bus: USER_CMD_BUS  NonVirtualBus=on
  Constant{,1,3..4} (4 alike) : Constant  Value=0  OutDataTypeStr=boolean
  Constant2 : Constant  OutDataTypeStr=boolean
  User Cmds : Outport
  wires:
  Bus Creator/1 -> User Cmds/1
  Constant/1 -> Bus Creator/1  "SAMPLE"
  Constant1/1 -> Bus Creator/2  "TARE"
  Constant2/1 -> Bus Creator/3  "MSG_ENABLE"
  Constant3/1 -> Bus Creator/4  "OVERRIDE_ENABLE"
  Constant4/1 -> Bus Creator/5  "OVERRIDE_VALUE"

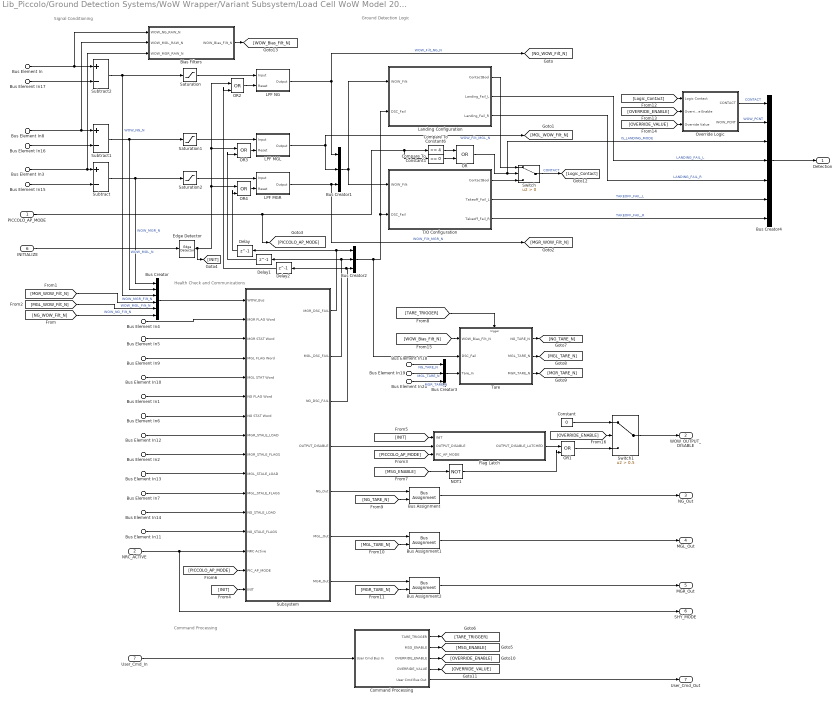
== system Lib_Piccolo/Ground Detection Systems/WoW Wrapper/Variant Subsystem/Load Cell WoW Model 20/WOW Module ==
  note: Command Processing
  note: Signal Conditioning
  note: Health Check and Communications
  note: Ground Detection Logic
  PICCOLO_AP_MODE : Inport  OutDataTypeStr=uint8
  NRC_ACTIVE : Inport  Port=2  OutDataTypeStr=boolean
  Bus Element In : Inport  Port=3  PortName=NG_In  Element=WOW_N
  Bus Element In1 : Inport  Port=3  PortName=NG_In  Element=DSC_FLAG_WORD
  Bus Element In6 : Inport  Port=3  PortName=NG_In  Element=DSC_STAT_WORD
  Bus Element In14 : Inport  Port=3  PortName=NG_In  Element=STALE_LOAD
  Bus Element In11 : Inport  Port=3  PortName=NG_In  Element=STALE_FLAGS
  Bus Element In17 : Inport  Port=3  PortName=NG_In  Element=TARE_N
  Bus Element In18 : Inport  Port=3  PortName=NG_In  Element=TARE_N
  Bus Element In8 : Inport  Port=4  PortName=MGL_In  Element=WOW_N
  Bus Element In9 : Inport  Port=4  PortName=MGL_In  Element=DSC_FLAG_WORD
  Bus Element In10 : Inport  Port=4  PortName=MGL_In  Element=DSC_STAT_WORD
  Bus Element In13 : Inport  Port=4  PortName=MGL_In  Element=STALE_LOAD
  Bus Element In7 : Inport  Port=4  PortName=MGL_In  Element=STALE_FLAGS
  Bus Element In16 : Inport  Port=4  PortName=MGL_In  Element=TARE_N
  Bus Element In19 : Inport  Port=4  PortName=MGL_In  Element=TARE_N
  Bus Element In4 : Inport  Port=5  PortName=MGR_In  Element=DSC_FLAG_WORD
  Bus Element In5 : Inport  Port=5  PortName=MGR_In  Element=DSC_STAT_WORD
  Bus Element In3 : Inport  Port=5  PortName=MGR_In  Element=WOW_N
  Bus Element In12 : Inport  Port=5  PortName=MGR_In  Element=STALE_LOAD
  Bus Element In2 : Inport  Port=5  PortName=MGR_In  Element=STALE_FLAGS
  Bus Element In15 : Inport  Port=5  PortName=MGR_In  Element=TARE_N
  Bus Element In20 : Inport  Port=5  PortName=MGR_In  Element=TARE_N
  INITIALIZE : Inport  Port=6  OutDataTypeStr=boolean
  User_Cmd_In : Inport  Port=7  OutDataTypeStr=Bus: USER_CMD_BUS
  Bias Filters : Subsystem
  Bus Assignment : BusAssignment  AssignedSignals=TARE_N
  Bus Assignment1 : BusAssignment  AssignedSignals=TARE_N
  Bus Assignment2 : BusAssignment  AssignedSignals=TARE_N
  Bus Creator : BusCreator  Inputs=6
  Bus Creator1 : BusCreator  Inputs=3
  Bus Creator2 : BusCreator  Inputs=3
  Bus Creator3 : BusCreator  Inputs=3
  Bus Creator4 : BusCreator  Inputs=7  OutDataTypeStr=Bus: DETECTION_BUS  NonVirtualBus=on
  Command Processing : Subsystem
  Compare To Constant1 : simulink/Logic and Bit Operations/Compare To Constant  relop===  const=0  OutDataTypeStr=uint8
  Compare To Constant6 : simulink/Logic and Bit Operations/Compare To Constant  relop=>=  const=4  OutDataTypeStr=uint8
  Constant : Constant  Value=0  OutDataTypeStr=boolean
  Delay : Delay  DelayLength=1
  Delay1 : Delay  DelayLength=1
  Delay2 : Delay  DelayLength=1
  Edge Detector : dspswit3/Edge Detector  InputProcessing=Columns as channels (frame based)
      settings: SourceProductName=DSP System Toolbox  SourceProductBaseCode=DS
  Flag Latch : Subsystem
  LPF MGL : Subsystem  mask{Cutoff=SensorModel.WOW.Cell.fc, Init=0}
      mask prompts: Cutoff "Cutoff Frequency [Hz]"; Init "Initial Condition"
  LPF MGR : Subsystem  mask{Cutoff=SensorModel.WOW.Cell.fc, Init=0}
      mask prompts: Cutoff "Cutoff Frequency [Hz]"; Init "Initial Condition"
  LPF NG : Subsystem  mask{Cutoff=SensorModel.WOW.Cell.fc, Init=0}
      mask prompts: Cutoff "Cutoff Frequency [Hz]"; Init "Initial Condition"
  Landing Configuration : Subsystem
  NOT1 : Logic  Operator=NOT  IconShape=distinctive  AllPortsSameDT=off  OutDataTypeStr=boolean
  OR{,1..4} (5 alike) : Logic  Operator=OR  IconShape=distinctive  AllPortsSameDT=off  OutDataTypeStr=boolean
  Override Logic : Subsystem
  Saturation : Saturate  UpperLimit=SensorModel.WOW.Cell.SaturationUpper  LowerLimit=SensorModel.WOW.Cell.SaturationLower
  Saturation1 : Saturate  UpperLimit=SensorModel.WOW.Cell.SaturationUpper  LowerLimit=SensorModel.WOW.Cell.SaturationLower
  Saturation2 : Saturate  UpperLimit=SensorModel.WOW.Cell.SaturationUpper  LowerLimit=SensorModel.WOW.Cell.SaturationLower
  Subsystem : Subsystem
  Subtract : Sum  Inputs=+-
  Subtract1 : Sum  Inputs=+-
  Subtract2 : Sum  Inputs=+-
  Switch : Switch  Criteria=u2 > Threshold
  Switch1 : Switch  Criteria=u2 > Threshold  Threshold=0.5
  T/O Configuration : Subsystem
  Tare : Subsystem
  Detection : Outport  OutDataTypeStr=Bus: DETECTION_BUS
  WOW_OUTPUT_DISABLE : Outport  Port=2  OutDataTypeStr=boolean
  NG_Out : Outport  Port=3  OutDataTypeStr=Bus: GEAR_OUTPUT_BUS
  MGL_Out : Outport  Port=4  OutDataTypeStr=Bus: GEAR_OUTPUT_BUS
  MGR_Out : Outport  Port=5  OutDataTypeStr=Bus: GEAR_OUTPUT_BUS
  SHY_MODE : Outport  Port=6  OutDataTypeStr=boolean
  User_Cmd_Out : Outport  Port=7  OutDataTypeStr=Bus: USER_CMD_BUS
  wires:
  Subtract/1 -> Bus Creator/1, Saturation2/1  "WOW_MGR_N"
  Switch/1 -> [Logic_Contact]  "CONTACT"
  OR/1 -> Bus Creator4/3, Switch/2  "IS_LANDING_MODE"
  T/O Configuration/1(ContactBool) -> Switch/3
  Compare To Constant1/1 -> OR/2
  LPF NG/1("Output ") -> [NG_WOW_Filt_N], Bus Creator1/1  "WOW_Filt_NG_N"
  Landing Configuration/1(ContactBool) -> Switch/1
  Subtract2/1 -> Bus Creator/3, Saturation/1  "WOW_NG_N"
  Subtract1/1 -> Bus Creator/2, Saturation1/1  "WOW_MGL_N"
  LPF MGL/1("Output ") -> [MGL_WOW_Filt_N], Bus Creator1/2  "WOW_Filt_MGL_N"
  Bus Creator1/1 -> T/O Configuration/1(WOW_Filt), Landing Configuration/1(WOW_Filt)
  Compare To Constant6/1 -> OR/1
  PICCOLO_AP_MODE/1 -> [PICCOLO_AP_MODE], Compare To Constant6/1, Compare To Constant1/1
  LPF MGR/1("Output ") -> [MGR_WOW_Filt_N], Bus Creator1/3  "WOW_Filt_MGR_N"
  Saturation2/1 -> LPF MGR/1("Input ")
  Saturation1/1 -> LPF MGL/1("Input ")
  Saturation/1 -> LPF NG/1("Input ")
  Bus Creator2/1 -> Tare/2(DSC_Fail), Landing Configuration/2(DSC_Fail), T/O Configuration/2(DSC_Fail)
  INITIALIZE/1 -> Edge Detector/1
  Subsystem/1(MGR_DSC_FAIL) -> Bus Creator2/1, Delay/1
  Subsystem/3(NG_DSC_FAIL) -> Delay2/1, Bus Creator2/3
  Subsystem/2(MGL_DSC_FAIL) -> Delay1/1, Bus Creator2/2
  Bus Creator/1 -> Subsystem/1(WOW_Bus)
  Bus Element In4/1 -> Subsystem/2(MGR FLAG Word)
  Bus Element In5/1 -> Subsystem/3(MGR STAT Word)
  Bus Element In9/1 -> Subsystem/4(MGL FLAG Word)
  Bus Element In10/1 -> Subsystem/5(MGL STAT Word)
  Bus Element In1/1 -> Subsystem/6(NG FLAG Word)
  Bus Element In6/1 -> Subsystem/7(NG STAT Word)
  NRC_ACTIVE/1 -> SHY_MODE/1, Subsystem/14(NRC Active)
  Subsystem/5(NG_Out) -> Bus Assignment/1
  Subsystem/6(MGL_Out) -> Bus Assignment1/1
  Subsystem/7(MGR_Out) -> Bus Assignment2/1
  [MGR_WOW_Filt_N] -> Bus Creator/4  "WOW_MGR_Filt_N"
  [MGL_WOW_Filt_N] -> Bus Creator/5  "WOW_MGL_Filt_N"
  [NG_WOW_Filt_N] -> Bus Creator/6  "WOW_NG_Filt_N"
  Edge Detector/1 -> [INIT], OR2/1, OR3/1, OR4/1
  OR2/1 -> LPF NG/2(Reset)
  OR3/1 -> LPF MGL/2(Reset)
  OR4/1 -> LPF MGR/2(Reset)
  Bus Element In12/1 -> Subsystem/8(MGR_STALE_LOAD)
  Bus Element In13/1 -> Subsystem/10(MGL_STALE_LOAD)
  Bus Element In14/1 -> Subsystem/12(NG_STALE_LOAD)
  [INIT] -> Subsystem/16(INIT)
  [INIT] -> Flag Latch/1(INIT)
  Subsystem/4(OUTPUT_DISABLE) -> Flag Latch/2(OUTPUT_DISABLE)
  [PICCOLO_AP_MODE] -> Flag Latch/3(PIC_AP_MODE)
  Flag Latch/1(OUTPUT_DISABLE_LATCHED) -> OR1/1
  [PICCOLO_AP_MODE] -> Subsystem/15(PIC_AP_MODE)
  Bus Element In11/1 -> Subsystem/13(NG_STALE_FLAGS)
  Bus Element In7/1 -> Subsystem/11(MGL_STALE_FLAGS)
  Bus Element In2/1 -> Subsystem/9(MGR_STALE_FLAGS)
  User_Cmd_In/1 -> Command Processing/1(User Cmd Bus In)
  [MSG_ENABLE] -> NOT1/1
  OR1/1 -> Switch1/3
  NOT1/1 -> OR1/2
  Bus Element In3/1 -> Bias Filters/3(WOW_MGR_RAW_N), Subtract/1
  Bus Element In15/1 -> Subtract/2
  Bus Element In16/1 -> Subtract1/2
  Bus Element In8/1 -> Bias Filters/2(WOW_MGL_RAW_N), Subtract1/1
  Bus Element In/1 -> Subtract2/1, Bias Filters/1(WOW_NG_RAW_N)
  Bus Element In17/1 -> Subtract2/2
  Command Processing/5(User Cmd Bus Out) -> User_Cmd_Out/1
  Command Processing/2(MSG_ENABLE) -> [MSG_ENABLE]
  Command Processing/1(TARE_TRIGGER) -> [TARE_TRIGGER]
  Bus Assignment/1 -> NG_Out/1
  Bus Assignment1/1 -> MGL_Out/1
  Bus Assignment2/1 -> MGR_Out/1
  [TARE_TRIGGER] -> Tare/Trigger
  Tare/1(NG_TARE_N) -> [NG_TARE_N]
  Tare/2(MGL_TARE_N) -> [MGL_TARE_N]
  Tare/3(MGR_TARE_N) -> [MGR_TARE_N]
  [NG_TARE_N] -> Bus Assignment/2
  [MGL_TARE_N] -> Bus Assignment1/2
  [MGR_TARE_N] -> Bus Assignment2/2
  Bus Element In18/1 -> Bus Creator3/1  "NG_TARE_N"
  Bus Element In19/1 -> Bus Creator3/2  "MGL_TARE_N"
  Bus Element In20/1 -> Bus Creator3/3  "MGR_TARE_N"
  Bus Creator3/1 -> Tare/3(Tare_In)
  Landing Configuration/2(Landing_Fail_L) -> Bus Creator4/4  "LANDING_FAIL_L"
  Landing Configuration/3(Landing_Fail_R) -> Bus Creator4/5  "LANDING_FAIL_R"
  T/O Configuration/2(Takeoff_Fail_L) -> Bus Creator4/6  "TAKEOFF_FAIL_L"
  T/O Configuration/3(Takeoff_Fail_R) -> Bus Creator4/7  "TAKEOFF_FAIL_R"
  Bus Creator4/1 -> Detection/1
  Command Processing/3(OVERRIDE_ENABLE) -> [OVERRIDE_ENABLE]
  Command Processing/4(OVERRIDE_VALUE) -> [OVERRIDE_VALUE]
  Override Logic/1(CONTACT) -> Bus Creator4/1  "CONTACT"
  [Logic_Contact] -> Override Logic/1(Logic Contact)
  [OVERRIDE_ENABLE] -> Override Logic/2(Override Enable)
  [OVERRIDE_VALUE] -> Override Logic/3(Override Value)
  Bias Filters/1(WOW_Bias_Filt_N) -> [WOW_Bias_Filt_N]
  [WOW_Bias_Filt_N] -> Tare/1(WOW_Bias_Filt_N)
  Override Logic/2(WOW_PCNT) -> Bus Creator4/2  "WOW_PCNT"
  [OVERRIDE_ENABLE] -> Switch1/2
  Constant/1 -> Switch1/1
  Switch1/1 -> WOW_OUTPUT_DISABLE/1
  Delay/1 -> OR4/2
  Delay1/1 -> OR3/2
  Delay2/1 -> OR2/2
